simulink model "hrir_headtracking"  (R2025a)
settings: Solver=VariableStepAuto  StartTime=0.0  StopTime=t_end  FixedStep=dt  RelTol=1e-3
undefined symbols (not defined in the file or in its folder): dspblkCoreblockFVToolHelper, gcbh, hrir_l, hrir_r, n_directions, psi0, q0
libraries: dspsnks4 x1, dspvision x1
settings Model: Creator=eoencue1  LastModifiedBy=eoencue1

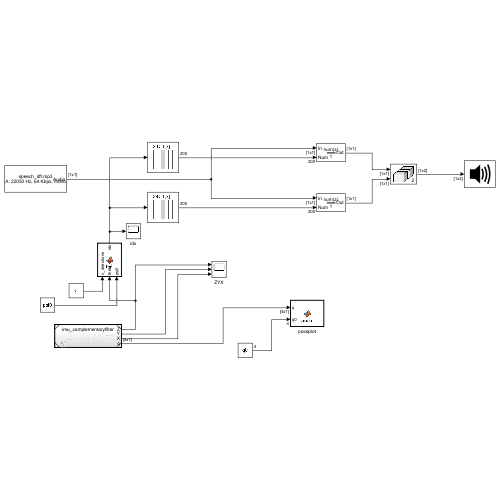
[thumbnail: Simulink's stored preview of the top-level diagram]
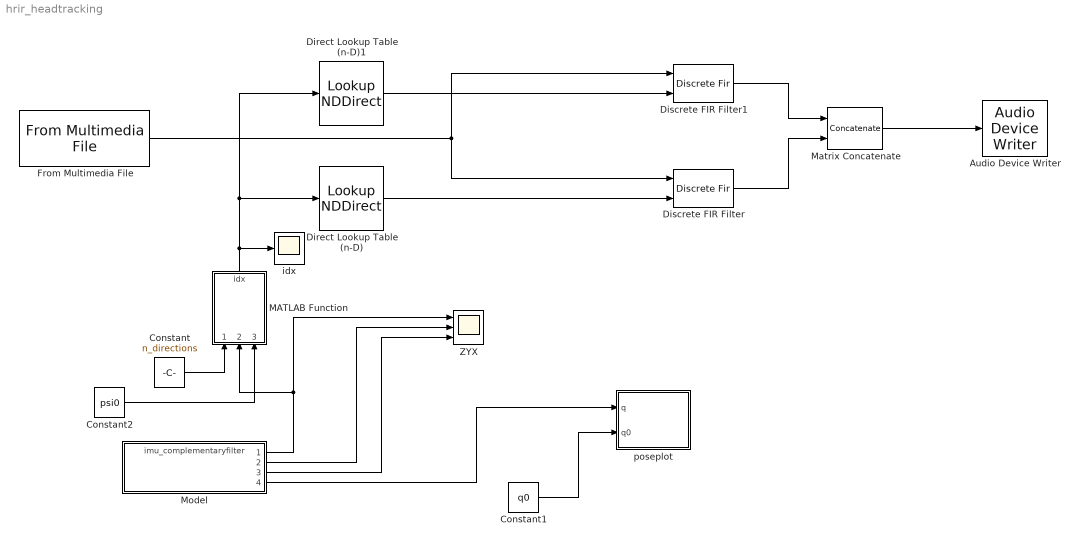
== system hrir_headtracking ==
  Audio Device Writer : dspsnks4/Audio Device Writer  Driver=DirectSound  Device=Default  InheritSampleRate=on  SampleRate=44100  BitDepth=16-bit integer  BufferSize=4096  NumBuffers=10  DefaultOutputChannelMapping=on  OutputChannelMapping=1:2  OutputNumUnderrunSamples=off  DriverIdx=1  DeviceWarnFlag=''
  Constant : Constant  Value=n_directions
  Constant1 : Constant  Value=q0
  Constant2 : Constant  Value=psi0
  Direct Lookup Table (n-D) : LookupNDDirect  InputsSelectThisObjectFromTable=Vector  Table=hrir_r
  Direct Lookup Table (n-D)1 : LookupNDDirect  InputsSelectThisObjectFromTable=Vector  Table=hrir_l
  Discrete FIR Filter : DiscreteFir  LoadFcn=dspblkCoreblockFVToolHelper(gcbh,'load');  CoefSource=Input port
      settings: CopyFcn=dspblkCoreblockFVToolHelper(gcbh,'copy');  DeleteFcn=dspblkCoreblockFVToolHelper(gcbh,'close');  ModelCloseFcn=dspblkCoreblockFVToolHelper(gcbh,'close');  PreSaveFcn=dspblkCoreblockFVToolHelper(gcbh,'presave');  PostSaveFcn=dspblkCoreblockFVToolHelper(gcbh,'postsave');  CloseFcn=dspblkCoreblockFVToolHelper(gcbh,'close');  InputPortMap=u0,u1
  Discrete FIR Filter1 : DiscreteFir  LoadFcn=dspblkCoreblockFVToolHelper(gcbh,'load');  CoefSource=Input port
      settings: CopyFcn=dspblkCoreblockFVToolHelper(gcbh,'copy');  DeleteFcn=dspblkCoreblockFVToolHelper(gcbh,'close');  ModelCloseFcn=dspblkCoreblockFVToolHelper(gcbh,'close');  PreSaveFcn=dspblkCoreblockFVToolHelper(gcbh,'presave');  PostSaveFcn=dspblkCoreblockFVToolHelper(gcbh,'postsave');  CloseFcn=dspblkCoreblockFVToolHelper(gcbh,'close');  InputPortMap=u0,u1
  From Multimedia File : dspvision/From Multimedia File  inputFilename=C:\Program Files\MATLAB\R2025a\toolbox\dsp\dsp\samples\speech_dft.mp3  readRange=[1 Inf]  loop=on  numPlays=inf  outputStreams=Audio only  videoDataType=single  audioDataType=double  inheritSampleTime=on  userDefinedSampleTime=dt  noAudioOutput=off  isIntensityVideo=off  fourcc=RGB  colorVideoFormat=Separate color signals  outputEOF=off  dataOrg=Column-major  audioFrameSize=1  computeAudioFrameSize=off  outSamplingMode=Sample based
      settings: LibrarySourceBlock=audiosources/From Multimedia File
  MATLAB Function : MATLAB Function  TreatAsAtomicUnit=on
  Matrix Concatenate : Concatenate  Mode=Multidimensional array  ConcatenateDimension=2
  Model : ModelReference  ModelNameDialog=imu_complementaryfilter.slx  SimulationMode=Normal  ModelReferenceVersion=1.43
  ZYX : Scope  NumInputPorts=3
      settings: ActiveDisplayYMinimum=-3.9246642098518087  ActiveDisplayYMaximum=3.920847570327485
  idx : Scope
      settings: ActiveDisplayYMinimum=-5.1249999999999982  ActiveDisplayYMaximum=56.125
  poseplot : MATLAB Function  TreatAsAtomicUnit=on
  wires:
  Model/1 -> ZYX/1, MATLAB Function/2(theta_z)
  From Multimedia File/1 -> Discrete FIR Filter1/1, Discrete FIR Filter/1
  Discrete FIR Filter/1 -> Matrix Concatenate/2
  MATLAB Function/1(idx) -> Direct Lookup Table (n-D)1/1, Direct Lookup Table (n-D)/1, idx/1
  Constant/1 -> MATLAB Function/1(n_directions)
  Discrete FIR Filter1/1 -> Matrix Concatenate/1
  Matrix Concatenate/1 -> Audio Device Writer/1
  Direct Lookup Table (n-D)/1 -> Discrete FIR Filter/2
  Direct Lookup Table (n-D)1/1 -> Discrete FIR Filter1/2
  Model/4 -> poseplot/1(q)
  Constant1/1 -> poseplot/2(q0)
  Model/2 -> ZYX/2
  Model/3 -> ZYX/3
  Constant2/1 -> MATLAB Function/3(psi0)

== matlab function hrir_headtracking/poseplot ==
  data: q input; q0 input
function pose(q, q0)
    persistent patch;
    coder.extrinsic("poseplot", "set", "drawnow", "gca", "xlabel", "ylabel", "zlabel", "view");

    q0inv = [q0(1); -q0(2:4)];
    q_rel = quaternion_mult(q, q0inv);
    if isempty(patch)
        patch = poseplot(quaternion([1 0 0 0]), "ENU");
        xlabel("X");
        ylabel("Y");
        zlabel("Z");
        ax = gca;
        set(ax, "XAxisLocation", "origin", "YAxisLocation", "origin");
        view(ax, -90, 60);
    end

    set(patch, "Orientation", quaternion(q_rel'));
    drawnow("limitrate");

== matlab function hrir_headtracking/MATLAB Function ==
  data: n_directions input; theta_z input; idx output; psi0 input
function idx = fcn(n_directions,theta_z,psi0)
    delta = (2*pi)/n_directions; 
    

    idx = mod(round(-(theta_z - psi0)/delta), n_directions);
